simulink model "MPPT_4x4"  (R2025b)
settings: Solver=ode23t  StartTime=0.0  StopTime=Tstop  MaxStep=1e-4  RelTol=1e-3
model workspace (MAT data in the model file):
  Cin = 0.00022
  Cin_esr = 0.05
  Cout = 0.00047
  G_tau = 0.001
  Gsched = [0 1000 1000 1000 1000 1000 1000 1000 1000 1000 1000 1000 1000 1000 1000 1000 1000]
  L = 0.00015
  RL = 0.01
  Rc = 0.05
  Rload = 10
  Tlog = 0.0005
  Tstop = 2
  byp_Goff = 4.4e-06
  byp_Ron = 0.012
  byp_Vf = 0.37
  mppt.alg = 1
  mppt.Tc = 5e-05
  mppt.Tmppt = 0.02
  mppt.Nper = 400
  mppt.Navg = 200
  mppt.Tsearch = 0.04
  mppt.Nper_s = 800
  mppt.Navg_s = 200
  mppt.dD = 0.005
  mppt.Dstart = 0.3
  mppt.Dmin = 0.05
  mppt.Dmax = 0.95
  mppt.Nwait = 3
  mppt.eps_inc = 0.3
  mppt.eps_di = 0.005
  mppt.Dlo = 0.3
  mppt.Dhi = 0.78
  mppt.dP_restart = 0.05
  mppt.restart_ref = 1
  mppt.T_rescan = 900
  mppt.Nmax = 64
  mppt.Drep = [0 0 0 0 0 0 0 0 0 0 0 0 0 0 0 0 0 0 0 0 0 0 0 0 0 0 0 0 0 0 0 0 0 0 0 0 0 0 0 0 0 0 0 0 0 0 0 0 0 0 0 0 0 0 0 0 0 0 0 0 0 0 0 0]
  mppt.Nrep = 0
  mppt.Nhold = 1
  mppt.local = [3 3 3 3 3 3 3 3]
  mppt.paper_end = 0
  mppt.vs_dDmax = 0.02
  mppt.vs_N = 0.0004
  mppt.vs_dDmin = 0.001
  mppt.vs_hold_dir = 1
  mppt.par_kmax = 3
  mppt.par_tol = 0.001
  mppt.par_h = 0.01
  mppt.chk_eps = 0.01
  mppt.chk_T = 1
  mppt.chk_d = 0.002
  mppt.chk_db = 0.0001
  mppt.chk_ramp = 0.001
  mppt.dir_range = 0
  mppt.dir_Voc_max = 183.2
  mppt.dir_Voc_min = 183.2
  mppt.dir_Isc_max = 36.44
  mppt.dir_Isc_min = 5.466
  mppt.dir_alpha = 0.15
  mppt.dir_beta = 0.7
  mppt.dir_eta = 1
  mppt.dir_Rload_min = 10
  mppt.dir_Rload_max = 10
  mppt.dir_Dlo_abs = 0.313660630165
  mppt.dir_Dhi_abs = 0.784552604435
  mppt.dir_c19 = 0.1
  mppt.dir_c20 = 0.2
  mppt.dir_eps_g = 0.03
  mppt.dir_eps_l = 0
  mppt.dir_Voc = 183.2
  mppt.dir_Isc = 36.44
  mppt.dir_kVmin = 0.333333333333
  mppt.dir_kImin = 0.333333333333
  mppt.dir_kVmax = 0.9
  mppt.dir_dcr = 0.0025
  mppt.eps_c = 0.02
  mppt.tau = 0.01
  mppt.delta_s = 0
  mppt.theta = 0.1
  mppt.c_corner = 1
  mppt.mg_on = 1
  mppt.mg_Voc = 183.2
  mppt.mg_Isc = 36.44
  mppt.pso_w = 0.4
  mppt.pso_c1 = 1.2
  mppt.pso_c2 = 1.6
  mppt.pso_D0 = [0.33 0.39 0.45 0.51 0.57 0.63 0.69 0.75]
  mppt.pso_dpert = 0.005
  mppt.pso_tol = 0.005
  mppt.pso_itmax = 8
  mppt.pso_reinit = 0
  mppt.pso_K1 = 17000
  mppt.pso_K2 = 0.05
  mppt.gwo_D0 = [0.34 0.42 0.5 0.58 0.66 0.74]
  mppt.gwo_itmax = 10
  mppt.gwo_tol = 0.005
  mppt.reset = 0
  mppt.rng_seed = 12345
  pv_EG = 1.11
  pv_Ir0 = 1000
  pv_Isc = 9.11
  pv_Ncell = 72
  pv_Ngrp = 24
  pv_Rs = 0.00441
  pv_T = 25
  pv_TIPH1 = 0.0005
  pv_TRS1 = 0
  pv_TXIS1 = 6.41
  pv_Tmeas = 25
  pv_Voc = 0.636111111111
  pv_n = 1
  sens.on = 0
  sens.bits = 12
  sens.FS = 3
  sens.kV = 0.015
  sens.kI = 0.056
  sens.eV = 0.004
  sens.oV = 0.0006
  sens.nV = 0.00033
  sens.eI = 0.0065
  sens.oI = 0.0112
  sens.nI = 0
  sens.adc_gain = 3
  sens.adc_off = 2
  sens.adc_inl = 1
  sens.adc_n = 0.42
  sens.seed = 1
libraries: ee_lib x97, nesl_utility x21, fl_lib x6
(part 1 of 4)
settings Model: Creator=soumy  LastModifiedBy=soumy

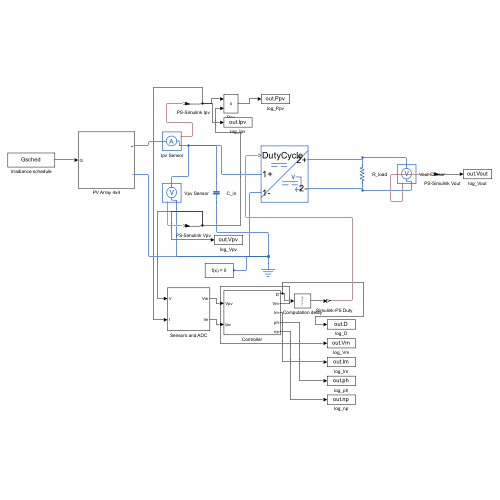
[thumbnail: Simulink's stored preview of the top-level diagram]
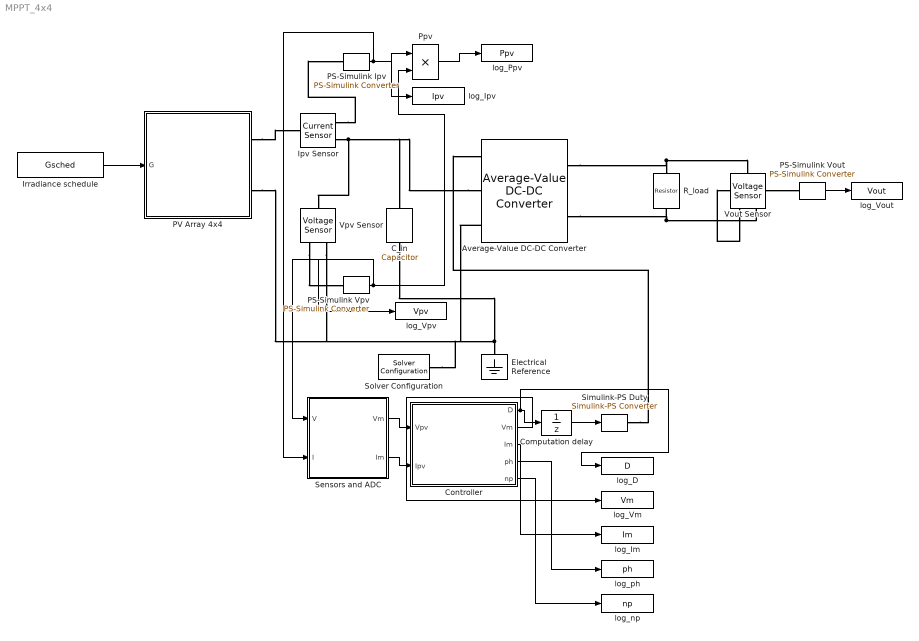
== system MPPT_4x4 ==
  Average-Value DC-DC Converter : ee_lib/Semiconductors & Converters/Converters/Average-Value DC-DC Converter  implementation_option=ee.enum.converters.implementation.averageValue  converter_type=ee.enum.converters.dcdctype.buckboost  control_option=ee.enum.converters.controlinput.dutycycle  efficiency_option=ee.enum.converters.efficiency.constant  efficiency_fixed=100  i_vec=[0, 2, 5] A  efficiency_vec=[90, 95, 98]  Lf=L H  Rl=RL Ohm  Cf=Cout F  Rc=Rc Ohm  iL_specify=off  iL_priority=High  iL=0 A  iL_nominal_specify=off  iL_nominal_value=1  iL_nominal_unit=A  vc_specify=off  vc_priority=High  vc=0 V  vc_nominal_specify=off  vc_nominal_value=1  vc_nominal_unit=V
      settings: InternalSimscapePortConfiguration="{\"Bottom\":[],\"Left\":[{\"id\":\"DutyCycle\",\"label\":\"DutyCycle\",\"type\":\"input\"},{\"id\":\"p1\",\"label\":\"1+\",\"type\":\"foundation.electrical.electrical\"},{\"id\":\"n1\",\"label\":\"1-\",\"type\":\"foundation.electrical.electrical\"}],\"Right\":[{\"id\":\"p2\",\"label\":\"2+\",\"type\":\"foundation.electrical.electrical\"},{\"id\":\"n2\",\"label\":\"2-\",\"type\":\"foundation.electrical.electrical\"}],\"Top\":[]}"
  C_in : fl_lib/Electrical/Electrical Elements/Capacitor  c=Cin F  r=Cin_esr Ohm  g=0 1/Ohm  i_specify=off  i_priority=None  i=0 A  i_nominal_specify=off  i_nominal_value=1  i_nominal_unit=A  v_specify=off  v_priority=None  v=0 V  v_nominal_specify=off  v_nominal_value=1  v_nominal_unit=V  vc_specify=off  vc_priority=High  vc=0 V  vc_nominal_specify=off  vc_nominal_value=1  vc_nominal_unit=V
  Computation delay : UnitDelay  InitialCondition=mppt.Dstart  SampleTime=mppt.Tc  HasFrameUpgradeWarning=on
  Controller : Subsystem
  Electrical Reference : fl_lib/Electrical/Electrical Elements/Electrical Reference
  Ipv Sensor : fl_lib/Electrical/Electrical Sensors/Current Sensor
  Irradiance schedule : FromWorkspace  VariableName=Gsched  Interpolate=off  OutputAfterFinalValue=Holding final value
  PS-Simulink Ipv : nesl_utility/PS-Simulink Converter  PhysicalDomain=network_engine_domain  SubClassName=ps_output  LeftPortType=input  RightPortType=output  PseudoPeriodic=off  Frequencies=[]  VectorFormat=inherit  Unit=A  AffineConversion=off
  PS-Simulink Vout : nesl_utility/PS-Simulink Converter  PhysicalDomain=network_engine_domain  SubClassName=ps_output  LeftPortType=input  RightPortType=output  PseudoPeriodic=off  Frequencies=[]  VectorFormat=inherit  Unit=V  AffineConversion=off
  PS-Simulink Vpv : nesl_utility/PS-Simulink Converter  PhysicalDomain=network_engine_domain  SubClassName=ps_output  LeftPortType=input  RightPortType=output  PseudoPeriodic=off  Frequencies=[]  VectorFormat=inherit  Unit=V  AffineConversion=off
  PV Array 4x4 : Subsystem
  Ppv : Product
  R_load : fl_lib/Electrical/Electrical Elements/Resistor  R=Rload Ohm  i_specify=off  i_priority=None  i=0 A  i_nominal_specify=off  i_nominal_value=1  i_nominal_unit=A  v_specify=off  v_priority=None  v=0 V  v_nominal_specify=off  v_nominal_value=1  v_nominal_unit=V
  Sensors and ADC : Subsystem
  Simulink-PS Duty : nesl_utility/Simulink-PS Converter  PhysicalDomain=network_engine_domain  SubClassName=ps_input  LeftPortType=input  RightPortType=output  PseudoPeriodic=off  Frequencies=[]  NoiseDistribution=none  NoiseParameters=[]  Unit=1  AffineConversion=off  FilteringAndDerivatives=zero  SimscapeFilterOrder=1  InputFilterTimeConstant=0.001  UdotUserProvided=0
  Solver Configuration : nesl_utility/Solver Configuration  PhysicalDomain=network_engine_domain  SubClassName=solver  LeftPortType=input  RightPortType=generic  Tones=[]  Harmonics=[]  SimulateNoise=off  Profile=off  UseLocalSampling=off  EnableSwitchedLinearOptims=on  FrequencyDomain=off  UseCCode=off  RelTol=0.001  AbsTol=0.001  MinStep=1e-09  ToWorkspace=off  RevertToSquareIcSolve=off  NumHomotopyIterations=100  PhasorMode=off  PhasorModeNumHarmonics=1  ConsistencySolver=NEWTON_XTOL_AFTER_FTOL  IndexReductionMethod=DerivativeReplacement  DoDC=off  ResidualTolerance=1e-09  ConsistencyTolSource=GLOBAL  ConsistencyAbsTol=0.001  ConsistencyRelTol=0.001  ConsistencyTolFactor=0.001  UseLocalSolver=off  LocalSolverChoice=NE_BACKWARD_EULER_ADVANCER  ResolveIndetEquations=on  FunctionEvalNumThread=1  LocalSolverSampleTime=0.001  DoFixedCost=off  MaxNonlinIter=3  MaxModeIter=2  ComputeImpulses=off  ImpulseIterations=2  LinearAlgebra=auto  LinearAlgebraNumThread=0  EquationFormulation=NE_TIME_EF  DelaysMemoryBudget=1024  AutomaticFiltering=on  FilteringTimeConstant=0.001  PartitionStorageMethod=AS_NEEDED  PartitionMemoryBudget=1024  PartitionMethod=ROBUST  MultibodyUseLocalSolver=off  MultibodyLocalSolverChoice=ODE1  MultibodyLocalSolverSampleTime=0.001
  Vout Sensor : fl_lib/Electrical/Electrical Sensors/Voltage Sensor
  Vpv Sensor : fl_lib/Electrical/Electrical Sensors/Voltage Sensor
  log_D : ToWorkspace  VariableName=D  SaveFormat=Timeseries  SampleTime=Tlog
  log_Im : ToWorkspace  VariableName=Im  SaveFormat=Timeseries  SampleTime=mppt.Tmppt
  log_Ipv : ToWorkspace  VariableName=Ipv  SaveFormat=Timeseries  SampleTime=Tlog
  log_Ppv : ToWorkspace  VariableName=Ppv  SaveFormat=Timeseries  SampleTime=Tlog
  log_Vm : ToWorkspace  VariableName=Vm  SaveFormat=Timeseries  SampleTime=mppt.Tmppt
  log_Vout : ToWorkspace  VariableName=Vout  SaveFormat=Timeseries  SampleTime=Tlog
  log_Vpv : ToWorkspace  VariableName=Vpv  SaveFormat=Timeseries  SampleTime=Tlog
  log_np : ToWorkspace  VariableName=np  SaveFormat=Timeseries  SampleTime=Tlog
  log_ph : ToWorkspace  VariableName=ph  SaveFormat=Timeseries  SampleTime=Tlog
  wires:
  Irradiance schedule/1 -> PV Array 4x4/1(G)
  PS-Simulink Ipv/1 -> Ppv/1, Sensors and ADC/2(I), log_Ipv/1
  PS-Simulink Vpv/1 -> Ppv/2, Sensors and ADC/1(V), log_Vpv/1
  Sensors and ADC/1(Vm) -> Controller/1(Vpv)
  Sensors and ADC/2(Im) -> Controller/2(Ipv)
  Controller/1(D) -> Computation delay/1, log_D/1
  Computation delay/1 -> Simulink-PS Duty/1
  Ppv/1 -> log_Ppv/1
  PS-Simulink Vout/1 -> log_Vout/1
  Controller/2(Vm) -> log_Vm/1
  Controller/3(Im) -> log_Im/1
  Controller/4(ph) -> log_ph/1
  Controller/5(np) -> log_np/1
  connections:
  PV Array 4x4/RConn1 -- Ipv Sensor/LConn1
  Average-Value DC-DC Converter/LConn2 -- Ipv Sensor/RConn2 -- C_in/LConn1 -- Vpv Sensor/LConn1
  C_in/RConn1 -- Vpv Sensor/RConn2 -- PV Array 4x4/RConn2 -- Average-Value DC-DC Converter/LConn3 -- Electrical Reference/LConn1 -- Solver Configuration/RConn1
  R_load/LConn1 -- Average-Value DC-DC Converter/RConn1 -- Vout Sensor/LConn1
  R_load/RConn1 -- Average-Value DC-DC Converter/RConn2 -- Vout Sensor/RConn2
  Vpv Sensor/RConn1 -- PS-Simulink Vpv/LConn1
  Ipv Sensor/RConn1 -- PS-Simulink Ipv/LConn1
  Vout Sensor/RConn1 -- PS-Simulink Vout/LConn1
  Simulink-PS Duty/RConn1 -- Average-Value DC-DC Converter/LConn1

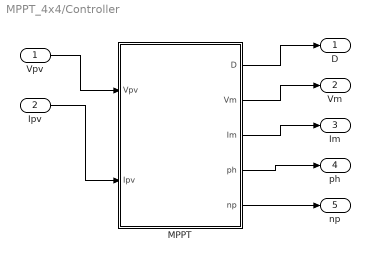
== system MPPT_4x4/Controller ==
  Vpv : Inport
  Ipv : Inport  Port=2
  MPPT : MATLAB Function  TreatAsAtomicUnit=on
  D : Outport
  Vm : Outport  Port=2
  Im : Outport  Port=3
  ph : Outport  Port=4
  np : Outport  Port=5
  wires:
  Vpv/1 -> MPPT/1(Vpv)
  Ipv/1 -> MPPT/2(Ipv)
  MPPT/1(D) -> D/1
  MPPT/2(Vm) -> Vm/1
  MPPT/3(Im) -> Im/1
  MPPT/4(ph) -> ph/1
  MPPT/5(np) -> np/1
